simulink model "simulinkFlow"  (R2023b)
settings: Solver=VariableStepAuto  StartTime=0.0  StopTime=10.0  RelTol=1e-3
libraries: simulink x1
settings Model: Creator=riccardoferrar  LastModifiedBy=mmazoespinosa

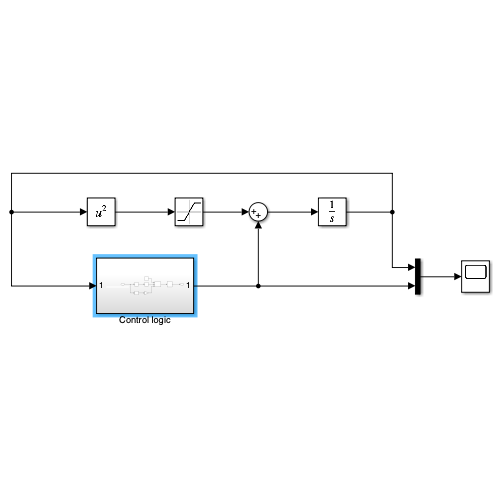
[thumbnail: Simulink's stored preview of the top-level diagram]
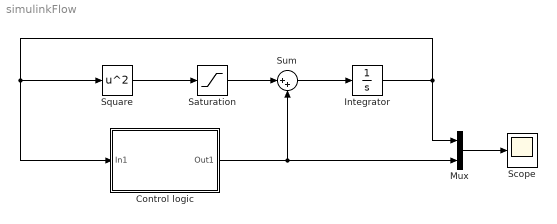
== system simulinkFlow ==
  Control logic : Subsystem
  Integrator : Integrator  InitialCondition=0.2
  Mux : Mux  Inputs=2
  Saturation : Saturate  UpperLimit=1  LowerLimit=-1
  Scope : Scope
  Square : Math  Operator=square
  Sum : Sum  Inputs=|++
  wires:
  Square/1 -> Saturation/1
  Saturation/1 -> Sum/1
  Sum/1 -> Integrator/1
  Integrator/1 -> Mux/1, Control logic/1(In1), Square/1
  Control logic/1(Out1) -> Mux/2, Sum/2
  Mux/1 -> Scope/1

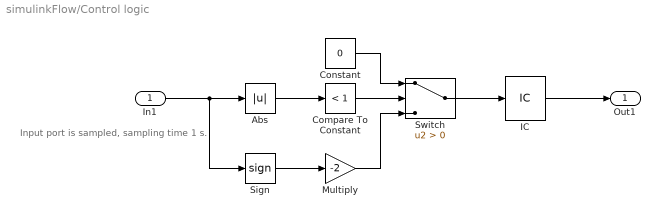
== system simulinkFlow/Control logic ==
  note: Input port is sampled, sampling time 1 s.
  In1 : Inport  SampleTime=1
  Abs : Abs  SaturateOnIntegerOverflow=off
  Compare To Constant : simulink/Logic and Bit Operations/Compare To Constant  relop=<  const=1  OutDataTypeStr=boolean
  Constant : Constant  Value=0
  IC : InitialCondition
  Multiply : Gain  Gain=-2
  Sign : Signum
  Switch : Switch  Criteria=u2 > Threshold  SaturateOnIntegerOverflow=off  InputSameDT=off
  Out1 : Outport  SampleTime=1
  wires:
  Multiply/1 -> Switch/3
  Sign/1 -> Multiply/1
  Switch/1 -> IC/1
  Abs/1 -> Compare To Constant/1
  In1/1 -> Sign/1, Abs/1
  Constant/1 -> Switch/1
  Compare To Constant/1 -> Switch/2
  IC/1 -> Out1/1
